simulink model "ev_bev_closed_loop_pi_tuned"  (R2026b)
settings: Solver=ode45  StopTime=25  MaxStep=0.02
settings Model: Creator=limaj  LastModifiedBy=limaj

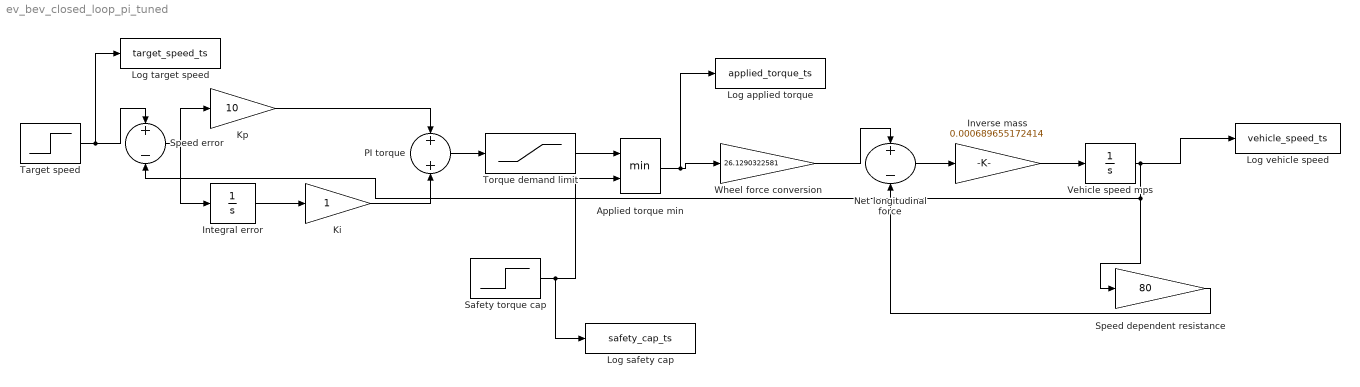
== system ev_bev_closed_loop_pi_tuned ==
  Applied torque min : MinMax  Inputs=2
  Integral error : Integrator
  Inverse mass : Gain  Gain=0.000689655172414
  Ki : Gain
  Kp : Gain  Gain=10
  Log applied torque : ToWorkspace  VariableName=applied_torque_ts  SaveFormat=Timeseries  SampleTime=-1
  Log safety cap : ToWorkspace  VariableName=safety_cap_ts  SaveFormat=Timeseries  SampleTime=-1
  Log target speed : ToWorkspace  VariableName=target_speed_ts  SaveFormat=Timeseries  SampleTime=-1
  Log vehicle speed : ToWorkspace  VariableName=vehicle_speed_ts  SaveFormat=Timeseries  SampleTime=-1
  Net longitudinal force : Sum  Inputs=+-
  PI torque : Sum
  Safety torque cap : Step  Time=12  InitialValue=200  FinalValue=0  SampleTime=0
  Speed dependent resistance : Gain  Gain=80
  Speed error : Sum  Inputs=+-
  Target speed : Step  Time=0.5  FinalValue=15  SampleTime=0
  Torque demand limit : Saturate  UpperLimit=200  LowerLimit=0
  Vehicle speed mps : Integrator
  Wheel force conversion : Gain  Gain=26.1290322581
  wires:
  Target speed/1 -> Speed error/1, Log target speed/1
  Speed error/1 -> Kp/1, Integral error/1
  Integral error/1 -> Ki/1
  Kp/1 -> PI torque/1
  Ki/1 -> PI torque/2
  PI torque/1 -> Torque demand limit/1
  Torque demand limit/1 -> Applied torque min/1
  Safety torque cap/1 -> Applied torque min/2, Log safety cap/1
  Applied torque min/1 -> Wheel force conversion/1, Log applied torque/1
  Wheel force conversion/1 -> Net longitudinal force/1
  Net longitudinal force/1 -> Inverse mass/1
  Inverse mass/1 -> Vehicle speed mps/1
  Vehicle speed mps/1 -> Speed error/2, Speed dependent resistance/1, Log vehicle speed/1
  Speed dependent resistance/1 -> Net longitudinal force/2
